simulink library "mssSimulink"  (R2024a)
settings: Solver=ode45  StartTime=0.0  StopTime=10.0  RelTol=1e-3
undefined symbols (not defined in the file): ABC, CN_data, CX_data, CY_data, D, G, Hoerner, K_supply, kt2ms, MA, magnitude, MRB, pathlength, RAO_Amp, RAO_Dir, RAO_Freq, RAO_Phase, RAO_Vel, RAO_yaw_back, RAO_yaw_quant, RAO_yaw_quantization_flag, rho_a, slcm, T_supply, table, vessel, vesselABC
libraries: $bdroot x99, simulink x13
(part 6 of 9)

== system mssSimulink/Hydrodynamics/Wave loads (U>0)/Wave loads U = U2 ==
  eta : Inport
  waves : Inport  Port=2
  U_idx : Inport  Port=3
  Abs : Abs
  Bus Selector : BusSelector  OutputSignals=Psi,Wavenum,Omega,Phase,Zeta_a
  Compare To Constant : simulink/Logic and Bit Operations/Compare To Constant  relop=<  const=0  OutDataTypeStr=uint8  ZeroCross=off
  Conversion : DataTypeConversion  OutDataTypeStr=double  SaturateOnIntegerOverflow=off  RndMeth=Floor
  D2R : Gain  Gain=pi/180
  "D2R " : Gain  Gain=pi/180
  Prelookup [0,180] : PreLookup  BreakpointsData=[0:10:180]  IndexSearchMethod=Evenly spaced points  BeginIndexSearchUsingPreviousIndexResult=on
  Product{,1..3} (4 alike) : Product  RndMeth=Zero
  R2D : Gain  Gain=180/pi
  Selector : Selector  InputPortWidth=6  IndexOptions=Index vector (dialog)  Indices=[6]  OutputSizes=1
  Sign : Signum
  Sum1 : Sum  Inputs=++|
  Sum2 : Sum  Inputs=++|
  Sum4 : Sum  Inputs=-+|
  Sum5 : Sum  Inputs=++|
  Wave loads for heading1 : Subsystem  mask(Force RAO){ForceRAO_Freq=vessel.forceRAO.w, WD_Freq=vessel.driftfrc.w, RAO_Vel=vessel.velocities, ForceRAO_Amp=vessel.forceRAO.amp, ForceRAO_Phase=vessel.forceRAO.phase, WD_Amp=vessel.driftfrc.amp, RAO_add_omega_0=on, RAO_add_omega_inf=on}
      mask prompts: ForceRAO_Freq "Vector of frequencies ForceRAO_Freq (rad/s)"; WD_Freq "Vector of frequencies WD_Freq (rad/s)"; RAO_Vel "Vector of velocities RAO_Vel (m/s)"; ForceRAO_Amp "6DOF Cell array with tables of Amplitudes ForceRAO_Amp"; ForceRAO_Phase "6DOF Cell array with tables of Phases ForceRAO_Phase (rad)"; WD_Amp "6DOF Cell array with tables of Amplitudes WD_Amp"; RAO_add_omega_0 "Add asymptotic RAO values for omega = 0"; RAO_add_omega_inf "Add asymptotic RAO values for omega = inf"
      mask help:
      | Calculate the 6 degrees-of-freedom (DOF) wave-frequency excitation forces tau_WF for a vessel from its Force Response Amplitude Operators (Force RAOs) and a sea state defined by a set of harmonic waves. The block takes the "Waves" bus from the MSS Waves block as input, as well as the vessel low-frequency (LF) motion in terms of the generalized position vector eta and mean surge velocity U. See help for details.
      |
      | Authors: Oyvind N. Smogeli and Thor I. Fossen, 2005-05-03
      mask init:
      | % use only nonzero increasing velocities, if zero element add eps
      | Nvel = length(RAO_Vel);
      | 
      | if Nvel == 1
      |     RAO_Vel = [0 1e10];   % use one data set for U=0 and one dummy set for u=1e10
      |     Nvel = 2;
      | end
      | 
      | for dof = 1:6
      |     TempFA{dof}  = ForceRAO_Amp{dof}(:,:,1:Nvel);
      |     TempFP{dof}  = ForceRAO_Phase{dof}(:,:,1:Nvel);
      | end
      | 
      | for dof = 1:3
      |     TempWA{dof}  = WD_Amp{dof}(:,:,1:Nvel);
      | end
      | 
      | clear ForceRAO_Amp ForceRAO_Phase WD_Amp WD_Phase
      | 
      | ForceRAO_Amp   = TempFA;
      | ForceRAO_Phase = TempFP;
      | WD_Amp         = TempWA;
      | 
      | % Add RAO values for zero frequency: use values for lowest given frequency
      | if RAO_add_omega_0 > 0
      | 	
      | 	if min(ForceRAO_Freq) > 0
      | 				
      | 		ForceRAO_Freq = [0 ForceRAO_Freq];
      | 		for dofno = 1:6
      | 			ForceRAO_Amp{dofno}   = [ForceRAO_Amp{dofno}(1,:,:);   ForceRAO_Amp{dofno}];
      | 			ForceRAO_Phase{dofno} = [ForceRAO_Phase{dofno}(1,:,:); ForceRAO_Phase{dofno}];
      |         end
      | 
      |     end
      |     
      | 	if min(WD_Freq) > 0
      |         
      | 		WD_Freq = [0 WD_Freq];
      | 		for dofno = 1:3
      | 			WD_Amp{dofno} = [WD_Amp{dofno}(1,:,:); WD_Amp{dofno}];
      | 		end        
      |         
      | 	end
      | 	
      | end
      | 
      | % Add RAO values for high frequency: use values for highest given frequency
      | maxfreq = 10;
      | if RAO_add_omega_inf > 0
      | 
      | 	if max(ForceRAO_Freq) < maxfreq
      | 			
      | 		newfreq = 2*max(ForceRAO_Freq) - ForceRAO_Freq(length(ForceRAO_Freq)-1);
      | 		
      | 		ForceRAO_Freq = [ForceRAO_Freq newfreq maxfreq];
      | 		for dofno = 1:6
      | 			ForceRAO_Amp{dofno}   = [ForceRAO_Amp{dofno};   zeros(2, 36, Nvel)];
      | 			ForceRAO_Phase{dofno} = [ForceRAO_Phase{dofno}; zeros(2, 36, Nvel)];
      | 		end
      | 		
      |     end
      | 
      | 	if max(WD_Freq) < maxfreq
      | 			
      | 		newfreq = 2*max(WD_Freq) - WD_Freq(length(WD_Freq)-1);
      | 		
      | 		WD_Freq = [WD_Freq newfreq maxfreq];
      | 		for dofno = 1:3
      | 			WD_Amp{dofno} = [WD_Amp{dofno}; zeros(2, 36, Nvel)];
      | 		end
      | 		
      |     end
      |     
      | end
      mask Help:
      | <b>Part of the Marine Systems Simulator: MSS</b><br>
      | <br>
      | Calculate the 6 degrees-of-freedom (DOF) wave-frequency excitation forces tau_WF
      | for a vessel from its Force Response Amplitude Operators (Force RAOs) and a sea
      | state defined by a set of harmonic waves. The block takes the &quot;Waves&quot; bus from
      | the MSS Waves block as input, as well as the vessel low-frequency (LF) motion in
      | terms of the generalized position vector eta and mean surge velocity U.<p>The Force RAOs are defined in terms of a
      | vector of frequencies (RAO_Freq), a vector of directions (RAO_Dir), a vector of
      | velocities (RAO_Dir), a 6DOF cell array of 3D matrices with amplitudes
      | (RAO_Amp), and a 6DOF cell array of 3D matrices with phases (RAO_Phase), which
      | are all input in the block mask. The first dimension of the 3D matrices
      | corresponds to the frequencies, the second to the directions, and the third to
      | the velocities, such that e.g. the amplitude amp in heave (DOF #3) for frequency
      | number n_f, direction number n_d and velocity number n_v can be found from a =
      | RAO_Amp{3}(n_f, n_d, n_v).</p>
      | <p><b>Inputs:</b></p>
      | <p>Waves:&nbsp;&nbsp;&nbsp;&nbsp;&nbsp;&nbsp;&nbsp;&nbsp;&nbsp;&nbsp;&nbsp; Bus
      | containing the following signals<br>
      | &nbsp;&nbsp;&nbsp; Zeta_a:&nbsp;&nbsp;&nbsp;&nbsp;&nbsp;&nbsp;&nbsp; Vector of harmonic wave amplitudes [m]<br>
      | &nbsp;&nbsp;&nbsp; Omega:&nbsp;&nbsp;&nbsp;&nbsp;&nbsp;&nbsp; Vector of harmonic wave frequencies [rad/s]<br>
      | &nbsp;&nbsp;&nbsp; Phase:&nbsp;&nbsp;&nbsp;&nbsp;&nbsp;&nbsp;&nbsp;&nbsp; Vector of harmonic wave phases (random) [rad]<br>
      | &nbsp;&nbsp;&nbsp; Wavenum:&nbsp;&nbsp;&nbsp; Vector of harmonic wave numbers [1/m]<br>
      | &nbsp;&nbsp;&nbsp; Psi:&nbsp;&nbsp;&nbsp;&nbsp;&nbsp;&nbsp;&nbsp;&nbsp;&nbsp;&nbsp;&nbsp;&nbsp;&nbsp; Vector of harmonic wave directions [rad]</p>
      | <p>eta_LF:&nbsp;&nbsp;&nbsp;&nbsp;&nbsp;&nbsp;&nbsp;&nbsp;&nbsp;&nbsp;&nbsp;
      | Generalized 6DOF n-frame low-frequency position vector [x (m), y (m), z (m),
      | theta (rad), phi (rad), psi (rad)]<br>
      | U:&nbsp;&nbsp;&nbsp;&nbsp;&nbsp;&nbsp;&nbsp;&nbsp;&nbsp;&nbsp;&nbsp;&nbsp;&nbsp;&nbsp;&nbsp;&nbsp;&nbsp;&nbsp;&nbsp;
      | Low-frequency (mean) surge velocity&nbsp; [m/s]</p>
      | <p><b>Outputs:</b></p>
      | <p>tau_WF:&nbsp;&nbsp;&nbsp;&nbsp;&nbsp;&nbsp;&nbsp;&nbsp;&nbsp; Generalized
      | 6DOF h-frame force vector [X (N), Y (N), Z (N), K (Nm), M (Nm), N (Nm)]</p>
      | <p><b>Model validity:</b></p>
      | <p>The validity of the block is dependent on the validity of the given
      | RAO data set.</p>
      | <p>A proper RAO to be used with this block should contain at least 1 velocity, 5
      | directions (e.g. 0, 45, 90, 135 and 180 degrees) and 10-20 frequencies, for all
      | 6 DOF (surge, sway, heave, roll, pitch, yaw).</p>
      | <p>The block performs linear interpolation in frequencies and directions, and
      | uses the data set for the velocity closest to the input velocity (i.e. 'nearest'
      | interpolation in velocity). If the block recieves an input wave frequency or relative
      | wave direction outside the span of the data vectors RAO_Freq or RAO_Dir
      | respectively, the simulation stops and an error is returned. This means that a well-defined
      | RAO must contain data for both 0 and 180 degrees, and for frequencies covering
      | the desired range of wave frequencies. If desired, asymptotic values can be
      | automatically added for zero and infinity frequency to avoid runtime errors if
      | the wave freqeuncy exceeds the values in RAO_Freq (see checkboxes in the mask). </p>
      | <p>IMPORTANT NOTE: The RAO theory upon which this block is based is in reality
      | only valid when the vessel low-frequency (h-frame) motion is a constant surge
      | velocity only, and the vessel is performing wave-frequency oscillations about
      | the steadily translating h-frame.This means that the outputs from the block when
      | manoeuvering -- i.e. changing the surge velocity and/or yaw angle -- must be
      | interpreted with some care. A jump in the output must be expected when changing
      | between two velocity data sets, and frequency warping expected when changing the
      | yaw angle (due to interpolation in the phase). It is therefore recommended to
      | use backlash on the input velocity to avoid transient switching, and a quantized
      | yaw angle with backlash. The latter will lead to jump in the ouput when the yaw
      | angle changes from one quantized value to another, but will give better results
      | when keeping within one quantizer interval. The quantized yaw angle with
      | backlash and velocity with backlash are available as options via checkboxes in
      | the mask. If either of these are activated, proper values for the yaw
      | quantization interval, yaw backlash width, and the the speed backlash width
      | respectively must be set. Typical values could be a yaw quantization interval of
      | 5 degrees, yaw backlash width of 1/4-1/5 of the quantization interval, and speed
      | backlash width of 1 m/s. To avoid the most rapid transients when switching
      | between data sets, output smoothing is available as an option in the mask. If
      | this is enabled, the output during a transent is rate limited according to the
      | fastest recorded signal rate during normal operation.</p>
      | <p><b>Example mask input:</b></p><p>
      | As an example, the format of the mask input for 2 velocities, 3 directions and 5
      | frequencies is as follows:<p>RAO_Freq = [f1 f2 f3 f4 f5]<br>
      | RAO_Dir = [d1 d2 d3]<br>
      | RAO_Vel = [v1 v2]<p>Surge:<br>
      | RAO_Amp{1}(:,:,1)&nbsp; = [a1_111 a1_121 a1_131; a1_211 a1_221 a1_231; a1_311
      | a1_321 a1_331; a1_411 a1_421 a1_431; a1_511 a1_521 a1_531]<br>
      | RAO_Amp{1}(:,:,2)&nbsp; = [a1_112 a1_122 a1_132; a1_212 a1_222 a1_232; a1_312
      | a1_322 a1_332; a1_412 a1_422 a1_432; a1_512 a1_522 a1_532]<br>
      | RAO_Phase{1}(:,:,1) = [p1_111 p1_121 p1_131; p1_211 p1_221 p1_231; p1_311 p1_321
      | p1_331; p1_411 p1_421 p1_431; p1_511 p1_521 p1_531]<br>
      | RAO_Phase{1}(:,:,2) = [p1_112 p1_122 p1_132; p1_212 p1_222 p1_232; p1_312 p1_322
      | p1_332; p1_412 p1_422 p1_432; p1_512 p1_522 p1_532]<p>Sway:<br>
      | RAO_Amp{2}(:,:,1)&nbsp; = [a2_111 a2_121 a2_131; a2_211 a2_221 a2_231; a2_311
      | a2_321 a2_331; a2_411 a2_421 a2_431; a2_511 a2_521 a2_531]<br>
      | RAO_Amp{2}(:,:,2)&nbsp; = [a2_112 a2_122 a2_132; a2_212 a2_222 a2_232; a2_312
      | a2_322 a2_332; a2_412 a2_422 a2_432; a2_512 a2_522 a2_532]<br>
      | RAO_Phase{2}(:,:,1) = [p2_111 p2_121 p2_131; p2_211 p2_221 p2_231; p2_311 p2_321
      | p2_331; p2_411 p2_421 p2_431; p2_511 p2_521 p2_531]<br>
      | RAO_Phase{2}(:,:,2) = [p2_112 p2_122 p2_132; p2_212 p2_222 p2_232; p2_312 p2_322
      | p2_332; p2_412 p2_422 p2_432; p2_512 p2_522 p2_532]<p>...<p>Yaw:<br>
      | RAO_Amp{6}(:,:,1)&nbsp; = [a6_111 a6_121 a6_131; a6_211 a6_221 a6_231; a6_311
      | a6_321 a6_331; a6_411 a6_421 a6_431; a6_511 a6_521 a6_531]<br>
      | RAO_Amp{6}(:,:,2)&nbsp; = [a6_112 a6_122 a6_132; a6_212 a6_222 a6_232; a6_312
      | a6_322 a6_332; a6_412 a6_422 a6_432; a6_512 a6_522 a6_532]<br>
      | RAO_Phase{6}(:,:,1) = [p6_111 p6_121 p6_131; p6_211 p6_221 p6_231; p6_311 p6_321
      | p6_331; p6_411 p6_421 p6_431; p6_511 p6_521 p6_531]<br>
      | RAO_Phase{6}(:,:,2) = [p6_112 p6_122 p6_132; p6_212 p6_222 p6_232; p6_312 p6_322
      | p6_332; p6_412 p6_422 p6_432; p6_512 p6_522 p6_532]<p>where now for example the
      | amplitude and phase in sway (DOF 2) for frequency f5, direction d3 and velocity
      | v1 are given by RAO_Amp{2}(5,3,1) = a2_531 and RAO_Phase{2}(5,3,1) = p2_531.<p>
      | <b>Copyright (C) NTNU 2005</b></p>
      | <p><b>Author:</b> Oyvind N. Smogeli, 2005-05-03</p>
  Wave loads for heading2 : Subsystem  mask(Force RAO){ForceRAO_Freq=vessel.forceRAO.w, WD_Freq=vessel.driftfrc.w, RAO_Vel=vessel.velocities, ForceRAO_Amp=vessel.forceRAO.amp, ForceRAO_Phase=vessel.forceRAO.phase, WD_Amp=vessel.driftfrc.amp, RAO_add_omega_0=on, RAO_add_omega_inf=on}
      mask prompts: ForceRAO_Freq "Vector of frequencies ForceRAO_Freq (rad/s)"; WD_Freq "Vector of frequencies WD_Freq (rad/s)"; RAO_Vel "Vector of velocities RAO_Vel (m/s)"; ForceRAO_Amp "6DOF Cell array with tables of Amplitudes ForceRAO_Amp"; ForceRAO_Phase "6DOF Cell array with tables of Phases ForceRAO_Phase (rad)"; WD_Amp "6DOF Cell array with tables of Amplitudes WD_Amp"; RAO_add_omega_0 "Add asymptotic RAO values for omega = 0"; RAO_add_omega_inf "Add asymptotic RAO values for omega = inf"
      mask help:
      | Calculate the 6 degrees-of-freedom (DOF) wave-frequency excitation forces Tau_WF for a vessel from its Force Response Amplitude Operators (Force RAOs) and a sea state defined by a set of harmonic waves. The block takes the "Waves" bus from the MSS Waves block as input, as well as the vessel low-frequency (LF) motion in terms of the generalized position vector eta_LF and mean surge velocity U. See help for details.
      |
      | Copyright (C) NTNU 2005
      | Author: Oyvind N. Smogeli, 2005-05-03
      mask init: same as mssSimulink/Hydrodynamics/Wave loads (U>0)/Wave loads U = U2/Wave loads for heading1
      mask Help:
      | <b>Part of the Marine Systems Simulator: MSS</b><br>
      | <br>
      | Calculate the 6 degrees-of-freedom (DOF) wave-frequency excitation forces Tau_WF
      | for a vessel from its Force Response Amplitude Operators (Force RAOs) and a sea
      | state defined by a set of harmonic waves. The block takes the &quot;Waves&quot; bus from
      | the MSS Waves block as input, as well as the vessel low-frequency (LF) motion in
      | terms of the generalized position vector eta_LF and mean surge velocity U.<p>The Force RAOs are defined in terms of a
      | vector of frequencies (RAO_Freq), a vector of directions (RAO_Dir), a vector of
      | velocities (RAO_Dir), a 6DOF cell array of 3D matrices with amplitudes
      | (RAO_Amp), and a 6DOF cell array of 3D matrices with phases (RAO_Phase), which
      | are all input in the block mask. The first dimension of the 3D matrices
      | corresponds to the frequencies, the second to the directions, and the third to
      | the velocities, such that e.g. the amplitude amp in heave (DOF #3) for frequency
      | number n_f, direction number n_d and velocity number n_v can be found from a =
      | RAO_Amp{3}(n_f, n_d, n_v).</p>
      | <p><b>Inputs:</b></p>
      | <p>Waves:&nbsp;&nbsp;&nbsp;&nbsp;&nbsp;&nbsp;&nbsp;&nbsp;&nbsp;&nbsp;&nbsp; Bus
      | containing the following signals<br>
      | &nbsp;&nbsp;&nbsp; Zeta_a:&nbsp;&nbsp;&nbsp;&nbsp;&nbsp;&nbsp;&nbsp; Vector of harmonic wave amplitudes [m]<br>
      | &nbsp;&nbsp;&nbsp; Omega:&nbsp;&nbsp;&nbsp;&nbsp;&nbsp;&nbsp; Vector of harmonic wave frequencies [rad/s]<br>
      | &nbsp;&nbsp;&nbsp; Phase:&nbsp;&nbsp;&nbsp;&nbsp;&nbsp;&nbsp;&nbsp;&nbsp; Vector of harmonic wave phases (random) [rad]<br>
      | &nbsp;&nbsp;&nbsp; Wavenum:&nbsp;&nbsp;&nbsp; Vector of harmonic wave numbers [1/m]<br>
      | &nbsp;&nbsp;&nbsp; Psi:&nbsp;&nbsp;&nbsp;&nbsp;&nbsp;&nbsp;&nbsp;&nbsp;&nbsp;&nbsp;&nbsp;&nbsp;&nbsp; Vector of harmonic wave directions [rad]</p>
      | <p>eta_LF:&nbsp;&nbsp;&nbsp;&nbsp;&nbsp;&nbsp;&nbsp;&nbsp;&nbsp;&nbsp;&nbsp;
      | Generalized 6DOF n-frame low-frequency position vector [x (m), y (m), z (m),
      | theta (rad), phi (rad), psi (rad)]<br>
      | U:&nbsp;&nbsp;&nbsp;&nbsp;&nbsp;&nbsp;&nbsp;&nbsp;&nbsp;&nbsp;&nbsp;&nbsp;&nbsp;&nbsp;&nbsp;&nbsp;&nbsp;&nbsp;&nbsp;
      | Low-frequency (mean) surge velocity&nbsp; [m/s]</p>
      | <p><b>Outputs:</b></p>
      | <p>tau_WF:&nbsp;&nbsp;&nbsp;&nbsp;&nbsp;&nbsp;&nbsp;&nbsp;&nbsp; Generalized
      | 6DOF h-frame force vector [X (N), Y (N), Z (N), K (Nm), M (Nm), N (Nm)]</p>
      | <p><b>Model validity:</b></p>
      | <p>The validity of the block is dependent on the validity of the given
      | RAO data set.</p>
      | <p>A proper RAO to be used with this block should contain at least 1 velocity, 5
      | directions (e.g. 0, 45, 90, 135 and 180 degrees) and 10-20 frequencies, for all
      | 6 DOF (surge, sway, heave, roll, pitch, yaw).</p>
      | <p>The block performs linear interpolation in frequencies and directions, and
      | uses the data set for the velocity closest to the input velocity (i.e. 'nearest'
      | interpolation in velocity). If the block recieves an input wave frequency or relative
      | wave direction outside the span of the data vectors RAO_Freq or RAO_Dir
      | respectively, the simulation stops and an error is returned. This means that a well-defined
      | RAO must contain data for both 0 and 180 degrees, and for frequencies covering
      | the desired range of wave frequencies. If desired, asymptotic values can be
      | automatically added for zero and infinity frequency to avoid runtime errors if
      | the wave freqeuncy exceeds the values in RAO_Freq (see checkboxes in the mask). </p>
      | <p>IMPORTANT NOTE: The RAO theory upon which this block is based is in reality
      | only valid when the vessel low-frequency (h-frame) motion is a constant surge
      | velocity only, and the vessel is performing wave-frequency oscillations about
      | the steadily translating h-frame.This means that the outputs from the block when
      | manoeuvering -- i.e. changing the surge velocity and/or yaw angle -- must be
      | interpreted with some care. A jump in the output must be expected when changing
      | between two velocity data sets, and frequency warping expected when changing the
      | yaw angle (due to interpolation in the phase). It is therefore recommended to
      | use backlash on the input velocity to avoid transient switching, and a quantized
      | yaw angle with backlash. The latter will lead to jump in the ouput when the yaw
      | angle changes from one quantized value to another, but will give better results
      | when keeping within one quantizer interval. The quantized yaw angle with
      | backlash and velocity with backlash are available as options via checkboxes in
      | the mask. If either of these are activated, proper values for the yaw
      | quantization interval, yaw backlash width, and the the speed backlash width
      | respectively must be set. Typical values could be a yaw quantization interval of
      | 5 degrees, yaw backlash width of 1/4-1/5 of the quantization interval, and speed
      | backlash width of 1 m/s. To avoid the most rapid transients when switching
      | between data sets, output smoothing is available as an option in the mask. If
      | this is enabled, the output during a transent is rate limited according to the
      | fastest recorded signal rate during normal operation.</p>
      | <p><b>Example mask input:</b></p><p>
      | As an example, the format of the mask input for 2 velocities, 3 directions and 5
      | frequencies is as follows:<p>RAO_Freq = [f1 f2 f3 f4 f5]<br>
      | RAO_Dir = [d1 d2 d3]<br>
      | RAO_Vel = [v1 v2]<p>Surge:<br>
      | RAO_Amp{1}(:,:,1)&nbsp; = [a1_111 a1_121 a1_131; a1_211 a1_221 a1_231; a1_311
      | a1_321 a1_331; a1_411 a1_421 a1_431; a1_511 a1_521 a1_531]<br>
      | RAO_Amp{1}(:,:,2)&nbsp; = [a1_112 a1_122 a1_132; a1_212 a1_222 a1_232; a1_312
      | a1_322 a1_332; a1_412 a1_422 a1_432; a1_512 a1_522 a1_532]<br>
      | RAO_Phase{1}(:,:,1) = [p1_111 p1_121 p1_131; p1_211 p1_221 p1_231; p1_311 p1_321
      | p1_331; p1_411 p1_421 p1_431; p1_511 p1_521 p1_531]<br>
      | RAO_Phase{1}(:,:,2) = [p1_112 p1_122 p1_132; p1_212 p1_222 p1_232; p1_312 p1_322
      | p1_332; p1_412 p1_422 p1_432; p1_512 p1_522 p1_532]<p>Sway:<br>
      | RAO_Amp{2}(:,:,1)&nbsp; = [a2_111 a2_121 a2_131; a2_211 a2_221 a2_231; a2_311
      | a2_321 a2_331; a2_411 a2_421 a2_431; a2_511 a2_521 a2_531]<br>
      | RAO_Amp{2}(:,:,2)&nbsp; = [a2_112 a2_122 a2_132; a2_212 a2_222 a2_232; a2_312
      | a2_322 a2_332; a2_412 a2_422 a2_432; a2_512 a2_522 a2_532]<br>
      | RAO_Phase{2}(:,:,1) = [p2_111 p2_121 p2_131; p2_211 p2_221 p2_231; p2_311 p2_321
      | p2_331; p2_411 p2_421 p2_431; p2_511 p2_521 p2_531]<br>
      | RAO_Phase{2}(:,:,2) = [p2_112 p2_122 p2_132; p2_212 p2_222 p2_232; p2_312 p2_322
      | p2_332; p2_412 p2_422 p2_432; p2_512 p2_522 p2_532]<p>...<p>Yaw:<br>
      | RAO_Amp{6}(:,:,1)&nbsp; = [a6_111 a6_121 a6_131; a6_211 a6_221 a6_231; a6_311
      | a6_321 a6_331; a6_411 a6_421 a6_431; a6_511 a6_521 a6_531]<br>
      | RAO_Amp{6}(:,:,2)&nbsp; = [a6_112 a6_122 a6_132; a6_212 a6_222 a6_232; a6_312
      | a6_322 a6_332; a6_412 a6_422 a6_432; a6_512 a6_522 a6_532]<br>
      | RAO_Phase{6}(:,:,1) = [p6_111 p6_121 p6_131; p6_211 p6_221 p6_231; p6_311 p6_321
      | p6_331; p6_411 p6_421 p6_431; p6_511 p6_521 p6_531]<br>
      | RAO_Phase{6}(:,:,2) = [p6_112 p6_122 p6_132; p6_212 p6_222 p6_232; p6_312 p6_322
      | p6_332; p6_412 p6_422 p6_432; p6_512 p6_522 p6_532]<p>where now for example the
      | amplitude and phase in sway (DOF 2) for frequency f5, direction d3 and velocity
      | v1 are given by RAO_Amp{2}(5,3,1) = a2_531 and RAO_Phase{2}(5,3,1) = p2_531.<p>
      | <b>Copyright (C) NTNU 2005</b></p>
      | <p><b>Author:</b> Oyvind N. Smogeli, 2005-05-03</p>
  "deg to 180/180  " : $bdroot/Utilities/Math Operations/deg to 180//180
  one : Constant
  "one " : Constant
  psi1 : Subsystem
  psi2 : Subsystem
  tau_WF : Outport
  tau_WD : Outport  Port=2
  wires:
  R2D/1 -> "deg to 180/180  "/1
  Selector/1 -> R2D/1
  Sum5/1 -> tau_WD/1
  waves/1 -> Bus Selector/1
  Sum1/1 -> tau_WF/1
  "D2R "/1 -> Wave loads for heading2/2(psi)
  D2R/1 -> Wave loads for heading1/2(psi)
  psi2/1(psi) -> "D2R "/1
  Conversion/1 -> psi1/1(k), Sum2/2
  Prelookup [0,180]/2 -> Sum4/1, Product1/1, Product3/1
  psi1/1(psi) -> D2R/1
  Compare To Constant/1 -> psi2/2(0 or 1), psi1/2(0 or 1)
  Sign/1 -> Compare To Constant/1
  Abs/1 -> Prelookup [0,180]/1
  "deg to 180/180  "/1 -> Sign/1, Abs/1
  Sum2/1 -> psi2/1(k)
  one/1 -> Sum2/1
  Prelookup [0,180]/1 -> Conversion/1
  Product2/1 -> Sum5/1
  Product3/1 -> Sum5/2
  Wave loads for heading1/2(tau_WD) -> Product2/2
  Sum4/1 -> Product2/1, Product/1
  "one "/1 -> Sum4/2
  Product1/1 -> Sum1/2
  Product/1 -> Sum1/1
  Wave loads for heading1/1(tau_WF) -> Product/2
  Bus Selector/5 -> Wave loads for heading2/7(Zeta_a), Wave loads for heading1/7(Zeta_a)  "<Zeta_a>"
  Bus Selector/4 -> Wave loads for heading2/6(Phase), Wave loads for heading1/6(Phase)  "<Phase>"
  Bus Selector/3 -> Wave loads for heading2/5(Omega), Wave loads for heading1/5(Omega)  "<Omega>"
  Bus Selector/2 -> Wave loads for heading2/4(wavenum), Wave loads for heading1/4(wavenum)  "<Wavenum>"
  Bus Selector/1 -> Wave loads for heading2/3(psi_wave), Wave loads for heading1/3(psi_wave)  "<Psi>"
  eta/1 -> Selector/1, Wave loads for heading1/1(eta), Wave loads for heading2/1(eta)
  Wave loads for heading2/2(tau_WD) -> Product3/2
  Wave loads for heading2/1(tau_WF) -> Product1/2
  U_idx/1 -> Wave loads for heading2/8(U), Wave loads for heading1/8(U_idx)

== system mssSimulink/Hydrodynamics/Wave loads for heading1/Wave component loop ==
  number of iterations : Inport
  Psi_r : Inport  Port=2
  Omega : Inport  Port=3
  Phase_tot : Inport  Port=4
  Zeta_a : Inport  Port=5
  U : Inport  Port=6
  "                " : Trigonometry
  Direct Lookup Table (n-D) Beta : LookupNDDirect  NumberOfTableDimensions=1  Table=vessel.headings
  Direct Lookup Table (n-D) Velocity : LookupNDDirect  NumberOfTableDimensions=1  Table=RAO_Vel
  For Iterator : ForIterator  ResetStates=reset  IterationSource=external  IterationVariableDataType=double
  Force RAO tables : Subsystem  mask(RAO table lookup){}
      mask help:
      | Perform 3D table lookup in 6DOF RAO amplitudes and phases, using the relative wave heading psi_r, wave frequency omega and vessel velocity vel as inputs. See documentation of the Motion RAO block or Force RAO block for details. A warning is issued if the input is outside the range spanned by the RAOs.
      |
      | Author: Oyvind N. Smogeli and Thor I. Fossen, 2005-05-03
  Memory1 : Memory  InitialCondition=[0 0 0 0 0 0]'  InheritSampleTime=on
  Memory2 : Memory  InitialCondition=[0 0 0 0 0 0]'  InheritSampleTime=on
  Prelookup1 : PreLookup  BreakpointsData=vessel.headings  OutputSelection=Index only  IndexSearchMethod=Evenly spaced points  BeginIndexSearchUsingPreviousIndexResult=on
  Prelookup2 : PreLookup  BreakpointsData=RAO_Vel  OutputSelection=Index only  IndexSearchMethod=Linear search  BeginIndexSearchUsingPreviousIndexResult=on
  Product1 : Product  SaturateOnIntegerOverflow=on  OutDataTypeStr=Inherit: Same as first input
  Product3 : Product  Inputs=3  SaturateOnIntegerOverflow=on  OutDataTypeStr=Inherit: Same as first input
  Product4 : Product  SaturateOnIntegerOverflow=on  OutDataTypeStr=Inherit: Same as first input
  Selector{2..5} (4 alike) : Selector  IndexOptions=Index vector (port)  Indices=[1 3]  OutputSizes=1
  Sum1 : Sum  Inputs=++|  SaturateOnIntegerOverflow=on
  Sum4 : Sum  Inputs=++|  SaturateOnIntegerOverflow=on
  Sum5 : Sum  Inputs=++|  SaturateOnIntegerOverflow=on
  WD RAO tables : Subsystem  mask(RAO table lookup){}
      mask help:
      | Perform 3D table lookup in 6DOF RAO amplitudes and phases, using the relative wave heading psi_r, wave frequency omega and vessel velocity vel as inputs. See documentation of the Motion RAO block or Force RAO block for details. A warning is issued if the input is outside the range spanned by the RAOs.
      |
      | Author: Oyvind N. Smogeli and Thor I. Fossen, 2005-05-03
  "[-inf inf] to [-pi pi] " : $bdroot/Utilities/Math Operations/[-inf inf] to [-pi pi]
  "[-pi pi] to [0 2pi]" : Subsystem  mask([-inf inf] to [-pi pi]){}
      mask help: Converts an angle in rad to (-pi pi)
  tau_WF : Outport
  tau_WD : Outport  Port=2
  wires:
  WD RAO tables/1(amp) -> Product3/1
  Force RAO tables/1(amp) -> Product4/1
  Force RAO tables/2(phase) -> Sum5/1
  Direct Lookup Table (n-D) Velocity/1 -> WD RAO tables/3(U), Force RAO tables/3(U)
  Prelookup2/1 -> Direct Lookup Table (n-D) Velocity/1
  Direct Lookup Table (n-D) Beta/1 -> WD RAO tables/1(beta), Force RAO tables/1(beta)
  Prelookup1/1 -> Direct Lookup Table (n-D) Beta/1
  "[-inf inf] to [-pi pi] "/1 -> "[-pi pi] to [0 2pi]"/1(x [-pi pi])
  For Iterator/1 -> Selector5/2, Selector4/2, Selector2/2, Selector3/2  "i=1:N"
  Selector2/1 -> WD RAO tables/2(w), Force RAO tables/2(w)  "omega"
  "[-pi pi] to [0 2pi]"/1(0<y<2pi) -> Prelookup1/1
  Product3/1 -> Sum1/1
  Memory1/1 -> Sum1/2
  Sum1/1 -> tau_WD/1, Memory1/1
  Product4/1 -> Product1/2
  "                "/1 -> Product1/1
  Selector3/1 -> "[-inf inf] to [-pi pi] "/1  "psi_r"
  Selector5/1 -> Sum5/2  "phase"
  Product1/1 -> Sum4/1
  Memory2/1 -> Sum4/2
  Sum4/1 -> tau_WF/1, Memory2/1
  number of iterations/1 -> For Iterator/1
  Omega/1 -> Selector2/1
  Psi_r/1 -> Selector3/1
  U/1 -> Prelookup2/1
  Phase_tot/1 -> Selector5/1
  Zeta_a/1 -> Selector4/1
  Sum5/1 -> "                "/1
  Selector4/1 -> Product3/3, Product3/2, Product4/2  "zeta_a"

== system mssSimulink/Marine craft models/CyberShipII/saturation ==
  tau : Inport
  Demux : Demux  Outputs=3
      settings: DisplayOption=none
  Mux1 : Mux  Inputs=3
  Saturation : Saturate  UpperLimit=2  LowerLimit=-2
  Saturation1 : Saturate  UpperLimit=1.5  LowerLimit=-1.5
  Saturation2 : Saturate  UpperLimit=1.5  LowerLimit=-1.5
  sat_tau : Outport  VectorParamsAs1DForOutWhenUnconnected=off
  wires:
  Mux1/1 -> sat_tau/1
  tau/1 -> Demux/1
  Demux/1 -> Saturation/1
  Demux/2 -> Saturation1/1
  Demux/3 -> Saturation2/1
  Saturation/1 -> Mux1/1
  Saturation1/1 -> Mux1/2
  Saturation2/1 -> Mux1/3

== system mssSimulink/Marine craft models/Mariner class cargo ship (2nd -order)/Ship model ==
  note: heading
      | angle
  rudder angle : Inport
  Integrator : Integrator
  Nomoto 2nd-order model : TransferFcn  Numerator=[K*T3 K]  Denominator=[T1*T2 (T1+T2) 1]
  heading angle : Outport  VectorParamsAs1DForOutWhenUnconnected=off
  heading rate : Outport  Port=2  VectorParamsAs1DForOutWhenUnconnected=off
  wires:
  rudder angle/1 -> Nomoto 2nd-order model/1
  Nomoto 2nd-order model/1 -> heading rate/1, Integrator/1  "heading rate"
  Integrator/1 -> heading angle/1

== system mssSimulink/Marine craft models/Tanker (1st-order)/Ship model ==
  note: heading
      | angle
  rudder angle : Inport
  " Nomoto time constant" : Gain  Gain=1/T_supply  SaturateOnIntegerOverflow=on  OutDataTypeStr=Inherit: Same as input  ParamDataTypeStr=Inherit: Same as input
  Integrator : Integrator
  Integrator1 : Integrator
  Nomoto gain constant : Gain  Gain=K_supply  SaturateOnIntegerOverflow=on  OutDataTypeStr=Inherit: Same as input  ParamDataTypeStr=Inherit: Same as input
  Sum : Sum  Inputs=|+-  InputSameDT=on  SaturateOnIntegerOverflow=on  OutDataTypeStr=Inherit: Same as first input
  heading angle : Outport  VectorParamsAs1DForOutWhenUnconnected=off
  heading rate : Outport  Port=2  VectorParamsAs1DForOutWhenUnconnected=off
  wires:
  Integrator1/1 -> heading angle/1
  Integrator/1 -> Sum/2, Integrator1/1, heading rate/1  "heading  rate"
  Nomoto gain constant/1 -> Sum/1
  rudder angle/1 -> Nomoto gain constant/1
  Sum/1 -> " Nomoto time constant"/1
  " Nomoto time constant"/1 -> Integrator/1

== system mssSimulink/Marine craft models/Tanker (2nd-order)/Ship model ==
  note: heading
      | angle
  rudder angle : Inport
  Integrator : Integrator
  Nomoto 2nd-order model : TransferFcn  Numerator=[K*T3 K]  Denominator=[T1*T2 (T1+T2) 1]
  heading angle : Outport  VectorParamsAs1DForOutWhenUnconnected=off
  heading rate : Outport  Port=2  VectorParamsAs1DForOutWhenUnconnected=off
  wires:
  rudder angle/1 -> Nomoto 2nd-order model/1
  Nomoto 2nd-order model/1 -> heading rate/1, Integrator/1  "heading rate"
  Integrator/1 -> heading angle/1

== system mssSimulink/Modelling/Control Surfaces/Fin//Rudder Machinery ==
  Angle Comm : Inport
  Gain : Gain  Gain=1/tc  SaturateOnIntegerOverflow=on  OutDataTypeStr=Inherit: Same as input  ParamDataTypeStr=Inherit: Same as input
  Integrator : Integrator
  Saturation : Saturate  UpperLimit=Dvmax  LowerLimit=-Dvmax
  Saturation1 : Saturate  UpperLimit=Dmax  LowerLimit=-Dmax
  Sum : Sum  Inputs=|+-  InputSameDT=on  SaturateOnIntegerOverflow=on  OutDataTypeStr=Inherit: Same as first input
  "Actual Ang. " : Outport  VectorParamsAs1DForOutWhenUnconnected=off
  wires:
  Angle Comm/1 -> Saturation1/1
  Saturation/1 -> Integrator/1
  Saturation1/1 -> Sum/1
  Integrator/1 -> "Actual Ang. "/1, Sum/2
  Sum/1 -> Gain/1
  Gain/1 -> Saturation/1

== system mssSimulink/Modelling/Control Surfaces/Rudder ==
  note: Lift
  note: Drag
  "Alpha_eff " : Inport
  Vrel : Inport  Port=2
  Constant1 : Constant  Value=CD0
  Math Function : Math  Operator=square  SignedPower=on
  Mux2 : Mux
  Product1 : Product  Inputs=**  InputSameDT=on  SaturateOnIntegerOverflow=on  OutDataTypeStr=Inherit: Same as first input
  Product2 : Product  InputSameDT=on  SaturateOnIntegerOverflow=on  OutDataTypeStr=Inherit: Same as first input
  Product4 : Product  InputSameDT=on  SaturateOnIntegerOverflow=on  OutDataTypeStr=Inherit: Same as first input
  Saturation : Saturate  UpperLimit=stall  LowerLimit=-stall
  Sum1 : Sum  Inputs=|++  InputSameDT=on  SaturateOnIntegerOverflow=on  OutDataTypeStr=Inherit: Same as first input
  "gain " : Gain  Gain=1/(0.9*pi*ar)  SaturateOnIntegerOverflow=on  OutDataTypeStr=Inherit: Same as input  ParamDataTypeStr=Inherit: Same as input
  gain 1 : Gain  Gain=dCL  SaturateOnIntegerOverflow=on  OutDataTypeStr=Inherit: Same as input  ParamDataTypeStr=Inherit: Same as input
  gain 2 : Gain  Gain=-1  SaturateOnIntegerOverflow=on  OutDataTypeStr=Inherit: Same as input  ParamDataTypeStr=Inherit: Same as input
  pi/(2*stall)2 : Gain  Gain=0.5*rho*A  SaturateOnIntegerOverflow=on  OutDataTypeStr=Inherit: Same as input  ParamDataTypeStr=Inherit: Same as input
  pi/(2*stall)6 : Gain  Gain=-(VCG-0.5*sp)  SaturateOnIntegerOverflow=on  OutDataTypeStr=Inherit: Same as input  ParamDataTypeStr=Inherit: Same as input
  pi/(2*stall)7 : Gain  Gain=-LCG  SaturateOnIntegerOverflow=on  OutDataTypeStr=Inherit: Same as input  ParamDataTypeStr=Inherit: Same as input
  "[XYKN]'" : Outport  VectorParamsAs1DForOutWhenUnconnected=off
  wires:
  Product1/1 -> pi/(2*stall)2/1
  Vrel/1 -> Product1/2, Product1/1
  Constant1/1 -> Sum1/2
  "gain "/1 -> Sum1/1
  Math Function/1 -> "gain "/1
  Sum1/1 -> Product4/1
  pi/(2*stall)2/1 -> Product2/2, Product4/2
  Product4/1 -> gain 2/1
  gain 2/1 -> Mux2/1
  Mux2/1 -> "[XYKN]'"/1
  pi/(2*stall)6/1 -> Mux2/3
  Product2/1 -> Mux2/2, pi/(2*stall)6/1, pi/(2*stall)7/1
  pi/(2*stall)7/1 -> Mux2/4
  gain 1/1 -> Product2/1, Math Function/1
  Saturation/1 -> gain 1/1
  "Alpha_eff "/1 -> Saturation/1

== system mssSimulink/Modelling/Control Surfaces/Rudder forces 4-DOF ==
  Lift : Inport
  Drag : Inport  Port=2
  Constant : Constant  Value=LCG
  Constant2 : Constant  Value=rr
  Gain : Gain  Gain=-1  SaturateOnIntegerOverflow=on  OutDataTypeStr=Inherit: Same as input  ParamDataTypeStr=Inherit: Same as input
  Gain1 : Gain  Gain=-1  SaturateOnIntegerOverflow=on  OutDataTypeStr=Inherit: Same as input  ParamDataTypeStr=Inherit: Same as input
  Product1 : Product  InputSameDT=on  SaturateOnIntegerOverflow=on  OutDataTypeStr=Inherit: Same as first input
  Product2 : Product  InputSameDT=on  SaturateOnIntegerOverflow=on  OutDataTypeStr=Inherit: Same as first input
  X : Outport  VectorParamsAs1DForOutWhenUnconnected=off
  Y : Outport  Port=2  VectorParamsAs1DForOutWhenUnconnected=off
  K : Outport  Port=3  VectorParamsAs1DForOutWhenUnconnected=off
  N : Outport  Port=4  VectorParamsAs1DForOutWhenUnconnected=off
  wires:
  Gain/1 -> X/1
  Drag/1 -> Gain/1
  Gain1/1 -> Product2/1, Product1/1
  Product2/1 -> K/1
  Constant2/1 -> Product2/2
  Lift/1 -> Y/1, Gain1/1
  Constant/1 -> Product1/2
  Product1/1 -> N/1

== system mssSimulink/Modelling/Control Surfaces/Stabilizer Fins forces 4-DOF ==
  Nf : Inport
  Tf : Inport  Port=2
  Constant : Constant  Value=FCG
  Constant1 : Constant  Value=sinB
  Constant2 : Constant  Value=rf
  Gain : Gain  Gain=-1  SaturateOnIntegerOverflow=on  OutDataTypeStr=Inherit: Same as input  ParamDataTypeStr=Inherit: Same as input
  Gain1 : Gain  Gain=-2  SaturateOnIntegerOverflow=on  OutDataTypeStr=Inherit: Same as input  ParamDataTypeStr=Inherit: Same as input
  Product : Product  Inputs=3  InputSameDT=on  SaturateOnIntegerOverflow=on  OutDataTypeStr=Inherit: Same as first input
  Product1 : Product  InputSameDT=on  SaturateOnIntegerOverflow=on  OutDataTypeStr=Inherit: Same as first input
  Product2 : Product  InputSameDT=on  SaturateOnIntegerOverflow=on  OutDataTypeStr=Inherit: Same as first input
  X : Outport  VectorParamsAs1DForOutWhenUnconnected=off
  Y : Outport  Port=2  VectorParamsAs1DForOutWhenUnconnected=off
  K : Outport  Port=3  VectorParamsAs1DForOutWhenUnconnected=off
  N : Outport  Port=4  VectorParamsAs1DForOutWhenUnconnected=off
  wires:
  Product1/1 -> Y/1
  Product/1 -> N/1
  Constant/1 -> Product/3
  Constant1/1 -> Product/1, Product1/2
  Nf/1 -> Product/2, Gain1/1, Product1/1
  Constant2/1 -> Product2/2
  Product2/1 -> K/1
  Gain1/1 -> Product2/1
  Tf/1 -> Gain/1
  Gain/1 -> X/1

== system mssSimulink/Modelling/Control Surfaces/Steady State Hydrofoil ==
  Ang : Inport
  "Vf " : Inport  Port=2
  Constant1 : Constant  Value=CD0
  Gain : Gain  Gain=0.5*rho*A  SaturateOnIntegerOverflow=on  OutDataTypeStr=Inherit: Same as input  ParamDataTypeStr=Inherit: Same as input
  Lookup Table CL(Ang) : Lookup  InputValues=AE  Table=CLAE  LookUpMeth=Interpolation-Use End Values  SaturateOnIntegerOverflow=off
  Math Function : Math  Operator=square  SignedPower=on
  Product{1,3,5..7} (5 alike) : Product  Inputs=**  InputSameDT=on  SaturateOnIntegerOverflow=on  OutDataTypeStr=Inherit: Same as first input
  Product2 : Product  InputSameDT=on  SaturateOnIntegerOverflow=on  OutDataTypeStr=Inherit: Same as first input
  Product4 : Product  InputSameDT=on  SaturateOnIntegerOverflow=on  OutDataTypeStr=Inherit: Same as first input
  Saturation : Saturate  UpperLimit=AM  LowerLimit=-AM
  Sum1 : Sum  Inputs=|++  InputSameDT=on  SaturateOnIntegerOverflow=on  OutDataTypeStr=Inherit: Same as first input
  Sum2 : Sum  Inputs=|++  InputSameDT=on  SaturateOnIntegerOverflow=on  OutDataTypeStr=Inherit: Same as first input
  Sum3 : Sum  Inputs=|-+  InputSameDT=on  SaturateOnIntegerOverflow=on  OutDataTypeStr=Inherit: Same as first input
  Trigonometric Function : Trigonometry  Operator=cos
  Trigonometric Function1 : Trigonometry
  "gain " : Gain  Gain=1/(0.9*pi*ar)  SaturateOnIntegerOverflow=on  OutDataTypeStr=Inherit: Same as input  ParamDataTypeStr=Inherit: Same as input
  Lift : Outport  VectorParamsAs1DForOutWhenUnconnected=off
  Drag : Outport  Port=2  VectorParamsAs1DForOutWhenUnconnected=off
  N : Outport  Port=3  VectorParamsAs1DForOutWhenUnconnected=off
  T : Outport  Port=4  VectorParamsAs1DForOutWhenUnconnected=off
  wires:
  Lookup Table CL(Ang)/1 -> Math Function/1, Product2/1
  Product4/1 -> Drag/1, Product5/1, Product6/1
  Gain/1 -> Product2/2, Product4/2
  Sum1/1 -> Product4/1
  Math Function/1 -> "gain "/1
  "gain "/1 -> Sum1/1
  Constant1/1 -> Sum1/2
  "Vf "/1 -> Product1/1, Product1/2
  Product1/1 -> Gain/1
  Product2/1 -> Lift/1, Product3/1, Product7/1
  Product3/1 -> Sum2/1
  Product5/1 -> Sum2/2
  Trigonometric Function/1 -> Product3/2, Product6/2
  Trigonometric Function1/1 -> Product5/2, Product7/2
  Sum2/1 -> N/1
  Product6/1 -> Sum3/1
  Product7/1 -> Sum3/2
  Sum3/1 -> T/1
  Saturation/1 -> Lookup Table CL(Ang)/1
  Ang/1 -> Saturation/1, Trigonometric Function1/1, Trigonometric Function/1

== system mssSimulink/Modelling/Environmental Loads/Force RAO ==
  eta : Inport
  U : Inport  Port=2
  Waves : Inport  Port=3
  Abs : Abs  SaturateOnIntegerOverflow=off
  Backlash : Backlash  BacklashWidth=RAO_speed_back
  Bus Selector : BusSelector  OutputSignals=Psi,Wavenum,Omega,Phase,Zeta_a
  Clock : Clock
  Omega range error : $bdroot/Utilities/Simulation tools/Signal range error  Values=RAO_Freq  message=Wave frequency outside range of RAO table
  Output smoothing flag : Constant  Value=RAO_smoothing_flag
  "Position phase " : $bdroot/Modelling/Environmental Loads/Utilities/Position phase
  Product1 : Product  Inputs=**  SaturateOnIntegerOverflow=on  OutDataTypeStr=Inherit: Same as first input
  Psi_r range error : $bdroot/Utilities/Simulation tools/Signal range error  Values=RAO_Dir  message=Relative wave direction outside range of RAO table
  "Signal smoothing " : $bdroot/Modelling/Environmental Loads/Utilities/Signal smoothing
  Speed lookup table : Lookup  InputValues=RAO_Vel  Table=RAO_Vel  LookUpMeth=Use Input Nearest  SaturateOnIntegerOverflow=off
  Speed quantizer flag : Constant  Value=RAO_speed_backlash_flag
  Sum : Sum  Inputs=-++  SaturateOnIntegerOverflow=on
  Switch1 : Switch  Threshold=0.5  SaturateOnIntegerOverflow=off  InputSameDT=off
  Switch2 : Switch  Threshold=0.5  SaturateOnIntegerOverflow=off  InputSameDT=off
  Wave component loop : Subsystem  TreatAsAtomicUnit=on
  Width : Width  DataType=int32
  "Yaw quantizer " : $bdroot/Modelling/Environmental Loads/Utilities/Yaw quantizer  quant_flag=RAO_yaw_quantization_flag  quant=RAO_yaw_quant  back=RAO_yaw_back
  "[-inf inf] to [-pi pi]" : $bdroot/Utilities/Math Operations/[-inf inf] to [-pi pi]
  yaw angle : Selector  InputPortWidth=6  IndexOptions=Index vector (dialog)  Indices=6  OutputSizes=1
  tau WF : Outport  VectorParamsAs1DForOutWhenUnconnected=off
  wires:
  Wave component loop/2(Tau rate) -> "Signal smoothing "/2
  "Signal smoothing "/1 -> Switch2/1
  Wave component loop/1(Tau WF) -> "Signal smoothing "/1, Switch2/3
  Switch2/1 -> tau WF/1
  Output smoothing flag/1 -> Switch2/2
  Abs/1 -> Psi_r range error/1
  "[-inf inf] to [-pi pi]"/1 -> Abs/1, Wave component loop/2(Psi_r)
  eta/1 -> yaw angle/1, "Position phase "/3
  Bus Selector/2 -> "Position phase "/2  "<Wavenum>"
  Bus Selector/4 -> Sum/3  "<Phase>"
  Waves/1 -> Bus Selector/1
  Product1/1 -> Sum/2
  Bus Selector/1 -> "Position phase "/1, "Yaw quantizer "/2  "<Psi>"
  Clock/1 -> Product1/2
  Bus Selector/3 -> Wave component loop/3(Omega), Omega range error/1, Width/1, Product1/1  "<Omega>"
  Sum/1 -> Wave component loop/4(Phase_tot)  "Phase_tot"
  Bus Selector/5 -> Wave component loop/5(Zeta_a)  "<Zeta_a>"
  Width/1 -> Wave component loop/1(number of iterations)
  U/1 -> Backlash/1, Switch1/3
  "Position phase "/1 -> Sum/1
  "Yaw quantizer "/1 -> "[-inf inf] to [-pi pi]"/1
  yaw angle/1 -> "Yaw quantizer "/1
  Speed quantizer flag/1 -> Switch1/2
  Backlash/1 -> Switch1/1
  Switch1/1 -> Speed lookup table/1
  Speed lookup table/1 -> Wave component loop/6(U)

== system mssSimulink/Modelling/Environmental Loads/Motion RAO ==
  eta LF : Inport
  U : Inport  Port=2
  Waves : Inport  Port=3
  6DOF rotation matrix in yaw : Subsystem
  Abs : Abs  SaturateOnIntegerOverflow=off
  Backlash : Backlash  BacklashWidth=RAO_speed_back
  Bus Selector : BusSelector  OutputSignals=Psi,Wavenum,Omega,Phase,Zeta_a
  Clock : Clock
  Omega range error : $bdroot/Utilities/Simulation tools/Signal range error  Values=RAO_Freq  message=Wave frequency outside range of RAO table
  Output smoothing : Subsystem
  "Position phase " : $bdroot/Modelling/Environmental Loads/Utilities/Position phase
  Product1 : Product  Inputs=**  SaturateOnIntegerOverflow=on  OutDataTypeStr=Inherit: Same as first input
  Psi_r range error : $bdroot/Utilities/Simulation tools/Signal range error  Values=RAO_Dir  message=Relative wave direction outside range of RAO table
  Speed lookup table : Lookup  InputValues=RAO_Vel  Table=RAO_Vel  LookUpMeth=Use Input Nearest  SaturateOnIntegerOverflow=off
  Speed quantizer flag : Constant  Value=RAO_speed_backlash_flag
  Sum : Sum  Inputs=-++  SaturateOnIntegerOverflow=on
  Switch1 : Switch  Threshold=0.5  SaturateOnIntegerOverflow=off  InputSameDT=off
  Wave component loop : Subsystem  TreatAsAtomicUnit=on
  Width : Width  DataType=int32
  "Yaw quantizer " : $bdroot/Modelling/Environmental Loads/Utilities/Yaw quantizer  quant_flag=RAO_yaw_quantization_flag  quant=RAO_yaw_quant  back=RAO_yaw_back
  "[-inf inf] to [-pi pi]" : $bdroot/Utilities/Math Operations/[-inf inf] to [-pi pi]
  yaw angle : Selector  InputPortWidth=6  IndexOptions=Index vector (dialog)  Indices=6  OutputSizes=1
  eta WF : Outport  VectorParamsAs1DForOutWhenUnconnected=off
  nu WF : Outport  Port=2  VectorParamsAs1DForOutWhenUnconnected=off
  nu_dot WF : Outport  Port=3  VectorParamsAs1DForOutWhenUnconnected=off
  wires:
  Output smoothing/1("eta_h WF ") -> 6DOF rotation matrix in yaw/2(V)
  Wave component loop/4(nu_dot rate) -> Output smoothing/4(nu_dot rate)
  Wave component loop/1(eta_h WF) -> Output smoothing/1(eta_h WF)
  Output smoothing/3(nu_dot WF) -> nu_dot WF/1
  Output smoothing/2(nu WF) -> nu WF/1
  eta LF/1 -> yaw angle/1, "Position phase "/3
  Bus Selector/2 -> "Position phase "/2  "<Wavenum>"
  Bus Selector/4 -> Sum/3  "<Phase>"
  Waves/1 -> Bus Selector/1
  Product1/1 -> Sum/2
  Bus Selector/1 -> "Position phase "/1, "Yaw quantizer "/2  "<Psi>"
  Clock/1 -> Product1/2
  yaw angle/1 -> 6DOF rotation matrix in yaw/1(psi), "Yaw quantizer "/1
  Bus Selector/3 -> Wave component loop/3(Omega), Width/1, Omega range error/1, Product1/1  "<Omega>"
  6DOF rotation matrix in yaw/1(R(psi)*V) -> eta WF/1
  Sum/1 -> Wave component loop/4(Phase_tot)  "Phase_tot"
  Bus Selector/5 -> Wave component loop/5(Zeta_a)  "<Zeta_a>"
  Width/1 -> Wave component loop/1(number of iterations)
  U/1 -> Backlash/1, Switch1/3
  Wave component loop/2(nu WF) -> Output smoothing/2("nu WF ")
  Wave component loop/3(nu_dot WF) -> Output smoothing/3("nu_dot WF ")
  Abs/1 -> Psi_r range error/1
  "Yaw quantizer "/1 -> "[-inf inf] to [-pi pi]"/1
  "[-inf inf] to [-pi pi]"/1 -> Wave component loop/2(Psi_r), Abs/1
  Speed quantizer flag/1 -> Switch1/2
  Backlash/1 -> Switch1/1
  Switch1/1 -> Speed lookup table/1
  Speed lookup table/1 -> Wave component loop/6(U)
  "Position phase "/1 -> Sum/1

== system mssSimulink/Modelling/Environmental Loads/Utilities ==
  Position phase : Subsystem  mask(Position Phase){}
      mask help: Calculate the phase delay due to the vessel LF position.
  RAO tables : Subsystem  mask(RAO table lookup){RAO_Freq=RAO_Freq, RAO_Dir=RAO_Dir, RAO_Vel=RAO_Vel, RAO_Amp=RAO_Amp, RAO_Phase=RAO_Phase}
      mask prompts: RAO_Freq "Vector of frequencies (rad/s)"; RAO_Dir "Vector of directions (rad)"; RAO_Vel "Vector of velocities (m/s)"; RAO_Amp "6DOF Cell array with tables of Amplitudes"; RAO_Phase "6DOF Cell array with tables of Phases (rad)"
      mask help:
      | Perform 3D table lookup in 6DOF RAO amplitudes and phases, using the relative wave heading psi_r, wave frequency omega and vessel velocity vel as inputs. See documentation of the Motion RAO block or Force RAO block for details. A warning is issued if the input is outside the range spanned by the RAOs.
      |
      | Copyright (C) NTNU 2005
      |
      | Author: Oyvind N. Smogeli, 2005-05-03
  Signal smoothing : Subsystem  mask(Signal smoothing){}
      mask help:
      | Rate limit the input signal according to the recorded maximum signal rate.
      |
      | For example, in order to remove switching transients from a velocity signal, input the acceleration signal as signal rate.
  Yaw quantizer : Subsystem  mask(Yaw quantizer){quant_flag=RAO_yaw_quantization_flag, quant=RAO_yaw_quant, back=RAO_yaw_back}
      mask prompts: quant_flag "Quantizer flag {0,1}"; quant "Quantizer interval [rad]"; back "Backlash width [rad]"
      mask help: Apply quantization and backlash to the yaw angle if desired, and calculate the wave direction relative to the vessel. If the quantizer flag is set to zero, the two outputs are equal.

== system mssSimulink/Modelling/Kinematics/6 DOF transformation ==
  note: Theta
  note: v
  note: omega
  eta : Inport
  nu : Inport  Port=2
  "Euler angles to rotation matrix " : $bdroot/Modelling/Kinematics/Euler angles to rotation matrix
  "Euler angles to attitude transformation matrix " : $bdroot/Modelling/Kinematics/Euler angles to attitude transformation matrix
  Mux : Mux  Inputs=2
  Product : Product  Inputs=**  Multiplication=Matrix(*)  SaturateOnIntegerOverflow=on  OutDataTypeStr=Inherit: Same as first input
  Product1 : Product  Inputs=**  Multiplication=Matrix(*)  SaturateOnIntegerOverflow=on  OutDataTypeStr=Inherit: Same as first input
  Selector : Selector  InputPortWidth=6  IndexOptions=Index vector (dialog)  Indices=[4 5 6]  OutputSizes=1
  Selector1 : Selector  InputPortWidth=6  IndexOptions=Index vector (dialog)  Indices=[1 2 3]  OutputSizes=1
  Selector2 : Selector  InputPortWidth=6  IndexOptions=Index vector (dialog)  Indices=[4 5 6]  OutputSizes=1
  J(eta)*nu : Outport  VectorParamsAs1DForOutWhenUnconnected=off
  wires:
  Selector/1 -> "Euler angles to rotation matrix "/1, "Euler angles to attitude transformation matrix "/1
  eta/1 -> Selector/1
  "Euler angles to rotation matrix "/1 -> Product/1
  nu/1 -> Selector1/1, Selector2/1
  Selector1/1 -> Product/2
  Selector2/1 -> Product1/2
  "Euler angles to attitude transformation matrix "/1 -> Product1/1
  Product/1 -> Mux/1
  Mux/1 -> J(eta)*nu/1
  Product1/1 -> Mux/2

== system mssSimulink/Modelling/Kinematics/Crab angle ==
  u : Inport
  v : Inport  Port=2
  Trigonometric Function : Trigonometry  Operator=atan2
  beta_c : Outport
  wires:
  v/1 -> Trigonometric Function/1
  Trigonometric Function/1 -> beta_c/1  "beta_c"
  u/1 -> Trigonometric Function/2

== system mssSimulink/Modelling/Kinematics/Euler angles to inverse rotation matrix ==
  theta : Inport
  Mux2 : Mux  Inputs=2
  Mux3 : Mux  Inputs=9
  R11 : Fcn  Expr=u(5)*u(6)
  R12 : Fcn  Expr=u(5)*u(3)
  R13 : Fcn  Expr=-u(2)
  "R21 " : Fcn  Expr=-u(4)*u(3)+u(1)*u(2)*u(6)
  R22 : Fcn  Expr=u(4)*u(6)+u(1)*u(2)*u(3)
  R23 : Fcn  Expr=u(1)*u(5)
  "R31 " : Fcn  Expr=u(1)*u(3)+u(4)*u(2)*u(6)
  R32 : Fcn  Expr=-u(1)*u(6)+u(4)*u(2)*u(3)
  R33 : Fcn  Expr=u(4)*u(5)
  Reshape 9x1->3x3 : Reshape  OutputDimensionality=Customize  OutputDimensions=[3,3]
  cos(theta) : Trigonometry  Operator=cos
  sin(theta) : Trigonometry
  inv(R) : Outport  InitialOutput=0  VectorParamsAs1DForOutWhenUnconnected=off
  wires:
  R33/1 -> Mux3/9
  R32/1 -> Mux3/6
  "R21 "/1 -> Mux3/2
  "R31 "/1 -> Mux3/3
  R12/1 -> Mux3/4
  R22/1 -> Mux3/5
  R13/1 -> Mux3/7
  R23/1 -> Mux3/8
  Mux2/1 -> R12/1, "R21 "/1, R11/1, "R31 "/1, R22/1, R23/1, R33/1, R13/1, R32/1
  theta/1 -> sin(theta)/1, cos(theta)/1
  cos(theta)/1 -> Mux2/2
  sin(theta)/1 -> Mux2/1
  Mux3/1 -> Reshape 9x1->3x3/1
  R11/1 -> Mux3/1
  Reshape 9x1->3x3/1 -> inv(R)/1
